simulink model "sm_robot_run_04_actuator"  (R2025a)
settings: Solver=ode15s  StartTime=0.0  StopTime=6*T_cg/4  MaxStep=1e-2  RelTol=1e-3  EnableMultiTasking=on
InitFcn:
  | d2r = pi/180;
  | if (~exist('T_cg'))
  |   sm_robot_run_4legs_param_def_load(bdroot)
  | end
values from neighbouring files (symbols this model uses):
  N = 100    [Extr_Data_Cam_Roller_Curve.m]
undefined symbols (not defined in the file or in its folder): bw, J, th_dot0
libraries: fl_lib x16, nesl_utility x9, batteryecm_lib x1, ee_lib x1
CloseFcn:
  | try,close(h1_sm_robot_run_04_actuator),end
  | clear h1_sm_robot_run_04_actuator
  | 
  | clear logsout_sm_robot_run_04_actuator
  | clear simlog_sm_robot_run_04_actuator
Description:
  | Robot Leg Actuator
  | 
  | Copyright 2012-2025 The MathWorks, Inc.
settings Model: Creator=Rick  LastModifiedBy=smiller
settings SolverCC: AlgebraicLoopSolver=TrustRegion
settings DataIOCC: LimitDataPoints=on  MaxDataPoints=10000  SaveFormat=Array  SignalLoggingSaveFormat=ModelDataLogs  ReturnWorkspaceOutputs=off  SignalLoggingName=logsout_sm_robot_run_04_actuator
settings OptimizationCC: ReuseModelBlockBuffer=off  ExpressionDepthLimit=2147483647.0  InitFltsAndDblsToZero=on  LifeSpan=inf
settings DebuggingCC: UnderspecifiedInitializationDetection=Classic  MergeDetectMultiDrivingBlocksExec=none  FcnCallInpInsideContextMsg=warning  UnconnectedInputMsg=warning  UnconnectedOutputMsg=warning  UnconnectedLineMsg=warning  StateNameClashWarn=warning  PregeneratedLibrarySubsystemCodeDiagnostic=none  SFUnexpectedBacktrackingDiag=warning  SFNoUnconditionalDefaultTransitionDiag=warning  SFExecutionAtInitializationDiag=none  ArithmeticOperatorsInVariantConditions=warning
settings HardwareCC: ProdBitPerPointer=32.0  ProdBitPerSizeT=32.0  ProdBitPerPtrDiffT=32.0  ProdLargestAtomicFloat=None  ProdIntDivRoundTo=Undefined  ProdEndianess=Unspecified  ProdWordSize=32.0  ProdHWDeviceType=32-bit Generic
settings ModelReferenceCC: EnableRefExpFcnMdlSchedulingChecks=on  PropagateSignalLabelsOutOfModel=off
settings SFSimCC: SimUseLocalCustomCode=off  CustomCodeUndefinedFunction=UseInterfaceOnly
settings RTWCC: RTWUseLocalCustomCode=off  GPUComputeCapability=3.5  DLArmComputeVersion=19.05
settings CodeAppCC: StateflowObjectComments=on
settings GRTTargetCC: TargetLangStandard=C89/C90 (ANSI)  CombineOutputUpdateFcns=off  GRTInterface=on
settings ConfigComp: CovMetricSettings=dw  CovSaveCumulativeToWorkspaceVar=on  CovSaveSingleToWorkspaceVar=on  CovExternalEMLEnable=off
settings SimscapeCC: SimscapeNormalizeSystem=off  SimscapeLogType=all  SimscapeLogSimulationStatistics=on  SimscapeLogName=simlog_sm_robot_run_04_actuator  SimscapeLogDataHistory=10000.0

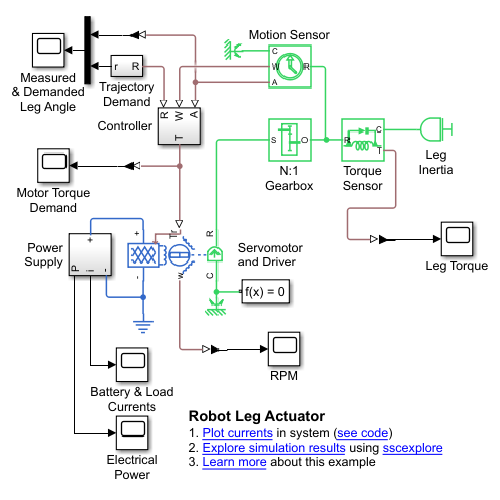
[thumbnail: Simulink's stored preview of the top-level diagram]
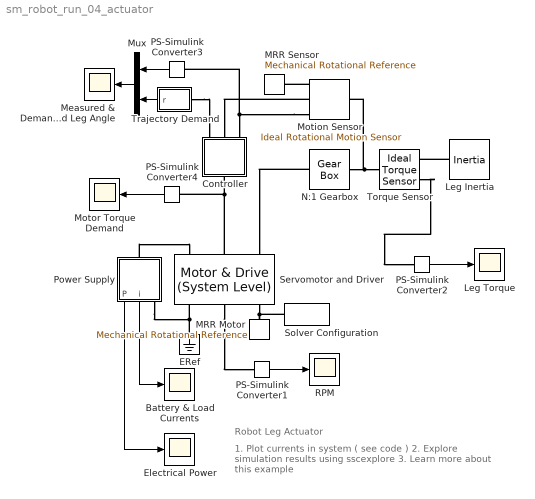
== system sm_robot_run_04_actuator ==
  note: Robot Leg Actuator
  note: 1. Plot currents in system ( see code )
      | 2. Explore simulation results using sscexplore
      | 3. Learn more about this example
  Battery & Load Currents : Scope
      settings: ActiveDisplayYMinimum=-1  ActiveDisplayYMaximum=1.5  DataLoggingVariableName=battery
  Controller : Subsystem
  ERef : fl_lib/Electrical/Electrical Elements/Electrical Reference
  Electrical Power : Scope
      settings: ActiveDisplayYMinimum=-20  ActiveDisplayYMaximum=30  DataLoggingVariableName=ScopeData4
  Leg Inertia : fl_lib/Mechanical/Rotational Elements/Inertia  inertia=J kg*m^2  num_ports=foundation.enum.numPorts2.one  w_specify=on  w_priority=High  w=th_dot0 deg/s  w_nominal_specify=off  w_nominal_value=1  w_nominal_unit=rad/s  t_specify=off  t_priority=None  t=0 N*m  t_nominal_specify=off  t_nominal_value=1  t_nominal_unit=N*m
  Leg Torque : Scope
      settings: TimeSpan=1.4  DataLoggingVariableName=ScopeData2
  MRR Motor : fl_lib/Mechanical/Rotational Elements/Mechanical Rotational Reference
  MRR Sensor : fl_lib/Mechanical/Rotational Elements/Mechanical Rotational Reference
  Measured & Demanded Leg Angle : Scope
      settings: ActiveDisplayYMinimum=-20  ActiveDisplayYMaximum=80
  Motion Sensor : fl_lib/Mechanical/Mechanical Sensors/Ideal Rotational Motion Sensor  reference=foundation.enum.MeasurementReference.difference  acceleration_port=false  velocity_port=true  position_port=true  wrap_angle=simscape.enum.onoff.off  offset=0 deg
  Motor Torque Demand : Scope
      settings: TimeSpan=1.4  ActiveDisplayYMinimum=-0.1  ActiveDisplayYMaximum=0.1  DataLoggingVariableName=ScopeData3
  Mux : Mux  Inputs=2
  N:1 Gearbox : fl_lib/Mechanical/Mechanisms/Gear Box  ratio=N  t_in_specify=off  t_in_priority=None  t_in=0 N*m  t_in_nominal_specify=off  t_in_nominal_value=1  t_in_nominal_unit=N*m  t_out_specify=off  t_out_priority=None  t_out=0 N*m  t_out_nominal_specify=off  t_out_nominal_value=1  t_out_nominal_unit=N*m
  PS-Simulink Converter1 : nesl_utility/PS-Simulink Converter  PhysicalDomain=network_engine_domain  SubClassName=ps_output  LeftPortType=input  RightPortType=output  PseudoPeriodic=off  Frequencies=[]  VectorFormat=1-D array  Unit=rpm  AffineConversion=off
  PS-Simulink Converter2 : nesl_utility/PS-Simulink Converter  PhysicalDomain=network_engine_domain  SubClassName=ps_output  LeftPortType=input  RightPortType=output  PseudoPeriodic=off  Frequencies=[]  VectorFormat=1-D array  Unit=N*m  AffineConversion=off
  PS-Simulink Converter3 : nesl_utility/PS-Simulink Converter  PhysicalDomain=network_engine_domain  SubClassName=ps_output  LeftPortType=input  RightPortType=output  PseudoPeriodic=off  Frequencies=[]  VectorFormat=1-D array  Unit=deg  AffineConversion=off
  PS-Simulink Converter4 : nesl_utility/PS-Simulink Converter  PhysicalDomain=network_engine_domain  SubClassName=ps_output  LeftPortType=input  RightPortType=output  PseudoPeriodic=off  Frequencies=[]  VectorFormat=1-D array  Unit=N*m  AffineConversion=off
  Power Supply : Subsystem
  RPM : Scope
      settings: ActiveDisplayYMinimum=-2000  ActiveDisplayYMaximum=4000
  Servomotor and Driver : ee_lib/Electromechanical/Motor & Drive (System Level)  torque_speed_param=1  overtorque_param=ee.enum.electromech.overtorque.no  T_t="[  0.13 0.115 0.1 0 ] N*m"  T_t_intermittent=[.36, .32, .28, 0] N*m  T_t_2D=[.09, .09, .09; .08, .08, .08; .07, .07, .07; 0, 0, 0] N*m  T_t_intermittent_2D=[.36, .36, .36; .32, .32, .32; .28, .28, .28; 0, 0, 0] N*m  w_t="[  0 2e+03 4e+03 4.1e3] rpm"  vdc_t=[6, 12, 24] V  torque_max=0.1 N*m  power_max=30 W  torque_max_intermittent=0.4 N*m  power_max_intermittent=120 W  time_overtorque=30 s  time_recover=60 s  Tc=0.01 s  EnableSwitch=simscape.enum.onoff.off  losses_param=1  eff=100  w_eff=3.75e+3 rpm  T_eff=0.08 N*m  Piron=0 W  Pbase=0 W  w_eff_vec=[-8000 -4000 0 4000 8000] rpm  T_eff_vec=[0 0.03 0.06 0.09] N*m  v_eff_vec=[100, 250, 400] V  losses_mat=[1.49 1.67 2.21 3.10; 0.42 0.69 1.14 2.03; 0.06 0.24 0.78 1.68; 0.42 0.69 1.14 2.03; 1.49 1.67 2.21 3.10] W  efficiency_mat=[95 95 95 95; 95 95 95 95; 95 95 95 95; 95 95 95 95; 95 95 95 95]  losses_mat_3D=ones(5, 4, 3) W  efficiency_mat_3D=95 * ones(5, 4, 3)  Res=1 Ohm  J=50 g*cm^2  lam=0 N*m/(rad/s)  speed0=th_dot0*N deg/s  faulted_specify=off  faulted_priority=None  faulted=0  faulted_nominal_specify=off  faulted_nominal_value=1  faulted_nominal_unit=1  isSwitchedOff_specify=off  isSwitchedOff_priority=None  isSwitchedOff=0  isSwitchedOff_nominal_specify=off  isSwitchedOff_nominal_value=1  isSwitchedOff_nominal_unit=1  torqueLimitContinuous_specify=off  torqueLimitContinuous_priority=None  torqueLimitContinuous=0 N*m  torqueLimitContinuous_nominal_specify=off  torqueLimitContinuous_nominal_value=1  torqueLimitContinuous_nominal_unit=N*m  alpha=3.93e-3 1/K  Tmeas=25 degC  Tmeas2=125 degC  losses_mat_T2=[1.49, 1.74, 2.49, 3.74; .42, .67, 1.42, 2.67; .06, .31, 1.06, 2.31; .42, .67, 1.42, 2.67; 1.49, 1.74, 2.49, 3.74] W  efficiency_mat_T2=[95, 95, 95, 95; 95, 95, 95, 95; 95, 95, 95, 95; 95, 95, 95, 95; 95, 95, 95, 95]  losses_mat_3D_T2=ones(5, 4, 3) W  efficiency_mat_3D_T2=95 * ones(5, 4, 3)  thermal_mass=100 J/K  initial_temperature=25 degC
  Solver Configuration : nesl_utility/Solver Configuration  PhysicalDomain=network_engine_domain  SubClassName=solver  LeftPortType=input  RightPortType=generic  Tones=[]  Harmonics=[]  SimulateNoise=off  Profile=off  UseLocalSampling=off  EnableSwitchedLinearOptims=on  FrequencyDomain=off  UseCCode=off  RelTol=0.001  AbsTol=1e-06  MinStep=1e-09  ToWorkspace=off  RevertToSquareIcSolve=off  NumHomotopyIterations=100  PhasorMode=off  PhasorModeNumHarmonics=1  ConsistencySolver=NEWTON_FTOL  IndexReductionMethod=DerivativeReplacement  DoDC=off  ResidualTolerance=1e-9  ConsistencyTolSource=GLOBAL  ConsistencyAbsTol=0.001  ConsistencyRelTol=0.001  ConsistencyTolFactor=0.001  UseLocalSolver=off  LocalSolverChoice=NE_BACKWARD_EULER_ADVANCER  ResolveIndetEquations=on  FunctionEvalNumThread=1  LocalSolverSampleTime=.001  DoFixedCost=off  MaxNonlinIter=12  MaxModeIter=2  ComputeImpulses=off  ImpulseIterations=2  LinearAlgebra=Sparse  LinearAlgebraNumThread=0  EquationFormulation=NE_TIME_EF  DelaysMemoryBudget=1024  AutomaticFiltering=on  FilteringTimeConstant=0.001  PartitionStorageMethod=AS_NEEDED  PartitionMemoryBudget=1024  PartitionMethod=FAST  MultibodyUseLocalSolver=off  MultibodyLocalSolverChoice=ODE1  MultibodyLocalSolverSampleTime=0.001
  Torque Sensor : fl_lib/Mechanical/Mechanical Sensors/Ideal Torque Sensor
  Trajectory Demand : Subsystem
  wires:
  PS-Simulink Converter2/1 -> Leg Torque/1
  PS-Simulink Converter1/1 -> RPM/1
  Trajectory Demand/1(r) -> Mux/2
  PS-Simulink Converter3/1 -> Mux/1
  Mux/1 -> Measured & Demanded Leg Angle/1
  PS-Simulink Converter4/1 -> Motor Torque Demand/1
  Power Supply/1(P) -> Electrical Power/1
  Power Supply/2(i) -> Battery & Load Currents/1
  connections:
  Power Supply/LConn1 -- Servomotor and Driver/LConn1
  Servomotor and Driver/RConn3 -- MRR Motor/LConn1 -- Solver Configuration/RConn1
  Torque Sensor/RConn2 -- PS-Simulink Converter2/LConn1
  Leg Inertia/LConn1 -- Torque Sensor/RConn1
  N:1 Gearbox/LConn1 -- Servomotor and Driver/LConn3
  N:1 Gearbox/RConn1 -- Torque Sensor/LConn1 -- Motion Sensor/LConn1
  Servomotor and Driver/LConn2 -- Controller/RConn1 -- PS-Simulink Converter4/LConn1
  Servomotor and Driver/RConn2 -- PS-Simulink Converter1/LConn1
  Motion Sensor/RConn1 -- MRR Sensor/LConn1
  Motion Sensor/RConn2 -- Controller/LConn2
  Trajectory Demand/LConn1 -- Controller/LConn1
  Motion Sensor/RConn3 -- PS-Simulink Converter3/LConn1 -- Controller/LConn3
  ERef/LConn1 -- Servomotor and Driver/RConn1 -- Power Supply/RConn1

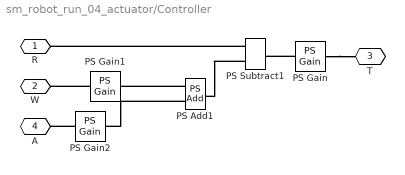
== system sm_robot_run_04_actuator/Controller ==
  PS Add1 : fl_lib/Physical Signals/Functions/PS Add
  PS Gain : fl_lib/Physical Signals/Functions/PS Gain  gain=bw*J/N
  PS Gain1 : fl_lib/Physical Signals/Functions/PS Gain  gain=1 (N*m)/(rad/s)
  PS Gain2 : fl_lib/Physical Signals/Functions/PS Gain  gain=1 (N*m)/(rad)
  PS Subtract1 : fl_lib/Physical Signals/Functions/PS Subtract
  R : PMIOPort  Side=Left
  W : PMIOPort  Port=2  Side=Left
  T : PMIOPort  Port=3  Side=Right
  A : PMIOPort  Port=4  Side=Left
  connections:
  PS Gain/LConn1 -- PS Subtract1/RConn1
  PS Gain/RConn1 -- T/RConn1
  PS Add1/LConn1 -- PS Gain1/RConn1
  PS Subtract1/LConn2 -- PS Add1/RConn1
  PS Add1/LConn2 -- PS Gain2/RConn1
  PS Subtract1/LConn1 -- R/RConn1
  PS Gain1/LConn1 -- W/RConn1
  PS Gain2/LConn1 -- A/RConn1

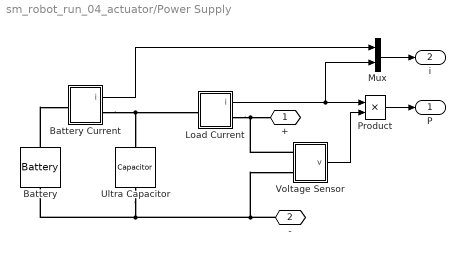
== system sm_robot_run_04_actuator/Power Supply ==
  Battery : batteryecm_lib/Battery  Vnom=24 V  prm_dir=1  R1_dis=2 Ohm  R1_ch=2 Ohm  R1=1 Ohm  prm_AH=2  AH=10 hr*A  V1=22 V  AH1=5 hr*A  prm_R2=1  R2=2e+03 Ohm  Tmeas=298.15 K  charge_measurement_port=simscape.enum.battery.enable.no  prm_dyn=1  Rp1=0.005 Ohm  tau1=30 s  Rp2=0.005 Ohm  tau2=30 s  Rp3=0.005 Ohm  tau3=30 s  Rp4=0.005 Ohm  tau4=30 s  Rp5=0.005 Ohm  tau5=30 s  prm_fade=1  N_fade=100  AH_fade=45 hr*A  R1_fade=2.02 Ohm  R1_ch_fade=2.02 Ohm  V1_fade=10.35 V  prm_age=1  prm_age_OCV=1  OCV_age=0.9  SOC_age=60  Tmeas_age=298.15 K  delta_time_age_vec=[0] d  temperature_age_vec=[273] K  OCV_scaling_age=2.2134e6  OCV_offset_age=1.632e6  temp_exp_age=0.515833569 V  t_exp_age=0.75  Vnom_T2=12 V  R1_T2=2.2 Ohm  R1_T2_dis=2.2 Ohm  R1_T2_ch=2.2 Ohm  V1_T2=11.4 V  R2_T2=2200 Ohm  Rp1_T2=0.005 Ohm  tau1_T2=30 s  Rp2_T2=0.005 Ohm  tau2_T2=30 s  Rp3_T2=0.005 Ohm  tau3_T2=30 s  Rp4_T2=0.005 Ohm  tau4_T2=30 s  Rp5_T2=0.005 Ohm  tau5_T2=30 s  Tmeas2=273.15 K  thermal_port=simscape.enum.thermaleffects.omit  thermal_mass=30000 J/K  i_specify=off  i_priority=None  i=0 A  i_nominal_specify=off  i_nominal_value=1  i_nominal_unit=A  v_specify=off  v_priority=None  v=0 V  v_nominal_specify=off  v_nominal_value=1  v_nominal_unit=V  charge_specify=on  charge_priority=High  charge=5 hr*A  charge_nominal_specify=off  charge_nominal_value=1  charge_nominal_unit=A*hr  num_cycles_specify=off  num_cycles_priority=High  num_cycles=0  num_cycles_nominal_specify=off  num_cycles_nominal_value=1  num_cycles_nominal_unit=1  temperature_specify=off  temperature_priority=High  temperature=298.15 K  temperature_nominal_specify=off  temperature_nominal_value=1  temperature_nominal_unit=K
  Battery Current : Subsystem
  Load Current : Subsystem
  Mux : Mux  Inputs=2
  Product : Product  RndMeth=Zero
  Ultra Capacitor : fl_lib/Electrical/Electrical Elements/Capacitor  c=1 F  r=1e-06 Ohm  g=0 1/Ohm  i_specify=off  i_priority=None  i=0 A  i_nominal_specify=off  i_nominal_value=1  i_nominal_unit=A  v_specify=off  v_priority=None  v=0 V  v_nominal_specify=off  v_nominal_value=1  v_nominal_unit=V  vc_specify=on  vc_priority=High  vc=22 V  vc_nominal_specify=off  vc_nominal_value=1  vc_nominal_unit=V
  Voltage Sensor : Subsystem
  + : PMIOPort  Side=Left
  - : PMIOPort  Port=2  Side=Right
  P : Outport  VectorParamsAs1DForOutWhenUnconnected=off
  i : Outport  Port=2  VectorParamsAs1DForOutWhenUnconnected=off
  wires:
  Load Current/1(i) -> Product/1, Mux/2
  Voltage Sensor/1(v) -> Product/2
  Product/1 -> P/1
  Battery Current/1(i) -> Mux/1
  Mux/1 -> i/1
  connections:
  -/RConn1 -- Voltage Sensor/LConn2 -- Battery/RConn1 -- Ultra Capacitor/RConn1
  Voltage Sensor/LConn1 -- +/RConn1 -- Load Current/RConn1
  Battery/LConn1 -- Battery Current/LConn1
  Battery Current/RConn1 -- Load Current/LConn1 -- Ultra Capacitor/LConn1

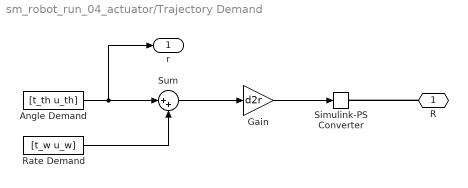
== system sm_robot_run_04_actuator/Trajectory Demand ==
  Angle Demand : FromWorkspace  VariableName=[t_th u_th]  ZeroCross=off  OutputAfterFinalValue=Holding final value
  Gain : Gain  Gain=d2r
  Rate Demand : FromWorkspace  VariableName=[t_w u_w]  ZeroCross=off  OutputAfterFinalValue=Holding final value
  Simulink-PS Converter : nesl_utility/Simulink-PS Converter  PhysicalDomain=network_engine_domain  SubClassName=ps_input  LeftPortType=input  RightPortType=output  PseudoPeriodic=off  Frequencies=[]  NoiseDistribution=none  NoiseParameters=[]  Unit=N*m  AffineConversion=off  FilteringAndDerivatives=zero  SimscapeFilterOrder=1  InputFilterTimeConstant=0.005  UdotUserProvided=[]
  Sum : Sum  Inputs=|++
  R : PMIOPort  Side=Left
  r : Outport  VectorParamsAs1DForOutWhenUnconnected=off
  wires:
  Gain/1 -> Simulink-PS Converter/1
  Sum/1 -> Gain/1
  Angle Demand/1 -> Sum/1, r/1
  Rate Demand/1 -> Sum/2
  connections:
  R/RConn1 -- Simulink-PS Converter/RConn1

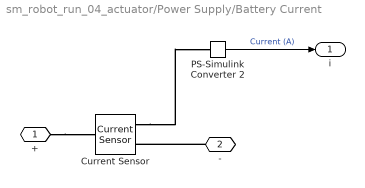
== system sm_robot_run_04_actuator/Power Supply/Battery Current ==
  Current Sensor : fl_lib/Electrical/Electrical Sensors/Current Sensor
  PS-Simulink Converter 2 : nesl_utility/PS-Simulink Converter  PhysicalDomain=network_engine_domain  SubClassName=ps_output  LeftPortType=input  RightPortType=output  PseudoPeriodic=off  Frequencies=[]  VectorFormat=1-D array  Unit=A  AffineConversion=off
  + : PMIOPort  Side=Left
  - : PMIOPort  Port=2  Side=Right
  i : Outport  VectorParamsAs1DForOutWhenUnconnected=off
  wires:
  PS-Simulink Converter 2/1 -> i/1  "Current (A)"
  connections:
  +/RConn1 -- Current Sensor/LConn1
  -/RConn1 -- Current Sensor/RConn2
  Current Sensor/RConn1 -- PS-Simulink Converter 2/LConn1

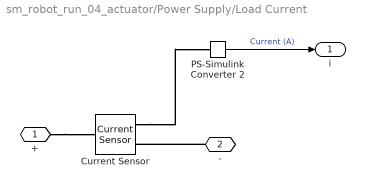
== system sm_robot_run_04_actuator/Power Supply/Load Current ==
  Current Sensor : fl_lib/Electrical/Electrical Sensors/Current Sensor
  PS-Simulink Converter 2 : nesl_utility/PS-Simulink Converter  PhysicalDomain=network_engine_domain  SubClassName=ps_output  LeftPortType=input  RightPortType=output  PseudoPeriodic=off  Frequencies=[]  VectorFormat=1-D array  Unit=A  AffineConversion=off
  + : PMIOPort  Side=Left
  - : PMIOPort  Port=2  Side=Right
  i : Outport  VectorParamsAs1DForOutWhenUnconnected=off
  wires:
  PS-Simulink Converter 2/1 -> i/1  "Current (A)"
  connections:
  Current Sensor/RConn1 -- PS-Simulink Converter 2/LConn1
  -/RConn1 -- Current Sensor/RConn2
  +/RConn1 -- Current Sensor/LConn1

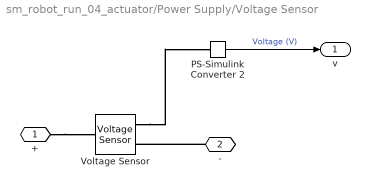
== system sm_robot_run_04_actuator/Power Supply/Voltage Sensor ==
  PS-Simulink Converter 2 : nesl_utility/PS-Simulink Converter  PhysicalDomain=network_engine_domain  SubClassName=ps_output  LeftPortType=input  RightPortType=output  PseudoPeriodic=off  Frequencies=[]  VectorFormat=1-D array  Unit=V  AffineConversion=off
  Voltage Sensor : fl_lib/Electrical/Electrical Sensors/Voltage Sensor
  + : PMIOPort  Side=Left
  - : PMIOPort  Port=2  Side=Left
  v : Outport  VectorParamsAs1DForOutWhenUnconnected=off
  wires:
  PS-Simulink Converter 2/1 -> v/1  "Voltage (V)"
  connections:
  +/RConn1 -- Voltage Sensor/LConn1
  -/RConn1 -- Voltage Sensor/RConn2
  Voltage Sensor/RConn1 -- PS-Simulink Converter 2/LConn1
